simulink model "nov12SimulinkAE4531"  (R2025a)
settings: Solver=VariableStepAuto  StartTime=0.0  StopTime=600  RelTol=1e-3
undefined symbols (not defined in the file or in its folder): A, B, C, D, u0
settings Model: Creator=rtydf  LastModifiedBy=rtydf

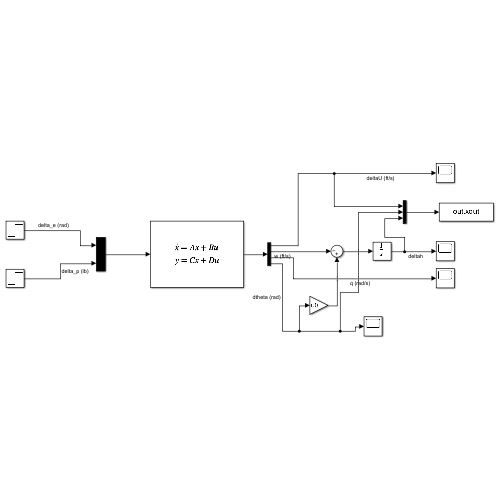
[thumbnail: Simulink's stored preview of the top-level diagram]
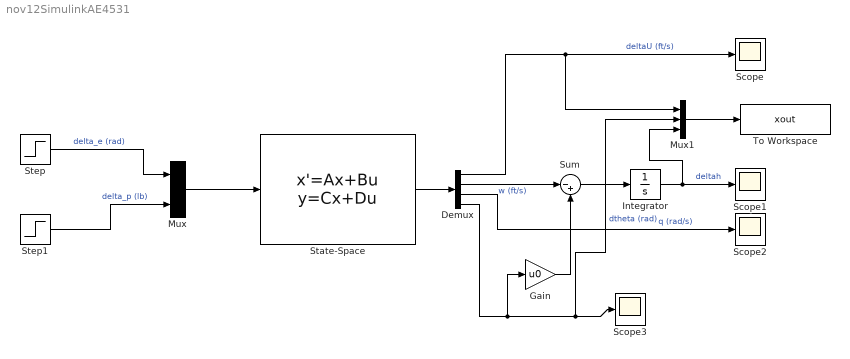
== system nov12SimulinkAE4531 ==
  Demux : Demux
  Gain : Gain  Gain=u0
  Integrator : Integrator
  Mux : Mux  Inputs=2
  Mux1 : Mux  Inputs=3
  Scope{,1..3} (4 alike) : Scope
      Scope settings: ActiveDisplayYMinimum=-11.2294123884496  ActiveDisplayYMaximum=12.358823598716622
      Scope1 settings: ActiveDisplayYMinimum=-60.53282145052799  ActiveDisplayYMaximum=544.795393054752
      Scope2 settings: ActiveDisplayYMinimum=-1  ActiveDisplayYMaximum=1  DataLoggingVariableName=ScopeData2
      Scope3 settings: ActiveDisplayYMinimum=-0.018364003296584906  ActiveDisplayYMaximum=0.020234049373339436  DataLoggingVariableName=ScopeData3
  State-Space : StateSpace  A=A  B=B  C=C  D=D  InitialCondition=[10; zeros(size(A,1)-1, 1)]
  Step : Step  After=0  SampleTime=0
  Step1 : Step  After=0  SampleTime=0
  Sum : Sum  Inputs=|-+
  To Workspace : ToWorkspace  VariableName=xout  SaveFormat=Timeseries  SampleTime=-1
  wires:
  State-Space/1 -> Demux/1
  Demux/1 -> Mux1/1, Scope/1  "deltaU (ft/s)"
  Demux/3 -> Scope2/1  "q (rad/s)"
  Demux/4 -> Gain/1, Mux1/2, Scope3/1  "dtheta (rad)"
  Mux/1 -> State-Space/1
  Step/1 -> Mux/1  "delta_e (rad)"
  Step1/1 -> Mux/2  "delta_p (lb)"
  Gain/1 -> Sum/2
  Demux/2 -> Sum/1  "w (ft/s)"
  Sum/1 -> Integrator/1
  Integrator/1 -> Mux1/3, Scope1/1  "deltah"
  Mux1/1 -> To Workspace/1
